simulink model "SimuNolineal"  (R2023b)
settings: Solver=VariableStepAuto  StartTime=0.0  StopTime=30  RelTol=1e-3
undefined symbols (not defined in the file): B, g, I, kd, ki, kp, kuf, kuf_0, lc, m, r
libraries: slpidlib x1
settings Model: Creator=sslan  LastModifiedBy=sslan

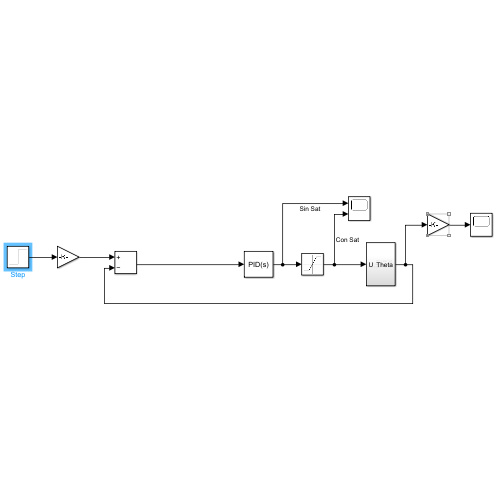
[thumbnail: Simulink's stored preview of the top-level diagram]
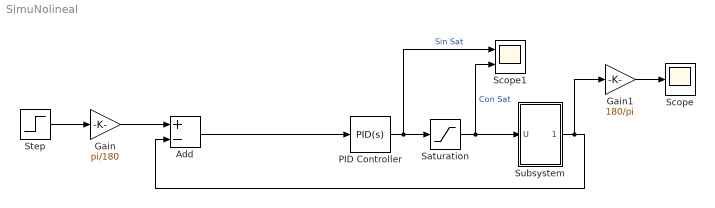
== system SimuNolineal ==
  Add : Sum  Inputs=+-
  Gain : Gain  Gain=pi/180
  Gain1 : Gain  Gain=180/pi
  PID Controller : slpidlib/PID Controller  Controller=PID  Form=Parallel  TimeDomain=Continuous-time  UseExternalTs=off  SampleTime=-1  IntegratorMethod=Forward Euler  FilterMethod=Forward Euler  ControllerParametersSource=internal  P=kp  I=ki  UseKiTs=off  D=kd  N=100  UseFilter=on  TunerSelectOption=Transfer Function Based (PID Tuner App)  InitialConditionSource=internal  InitialConditionForIntegrator=0  InitialConditionForFilter=0  DifferentiatorICPrevScaledInput=0  ExternalReset=none  TrackingMode=off  Kt=1  LimitOutput=off  SatLimitsSource=internal  UpperSaturationLimit=inf  LowerSaturationLimit=-inf  LinearizeAsGain=on  AntiWindupMode=none  Kb=1  LimitIntegrator=off  UpperIntegratorSaturationLimit=inf  LowerIntegratorSaturationLimit=-inf  POutMin=[]  POutMax=[]  IOutMin=[]  IOutMax=[]  DOutMin=[]  DOutMax=[]  NOutMin=[]  NOutMax=[]  SumOutMin=[]  SumOutMax=[]  SaturationOutMin=[]  SaturationOutMax=[]  PParamMin=[]  PParamMax=[]  IParamMin=[]  IParamMax=[]  DParamMin=[]  DParamMax=[]  NParamMin=[]  NParamMax=[]  KbParamMin=[]  KbParamMax=[]  KtParamMin=[]  KtParamMax=[]  KbOutMin=[]  KbOutMax=[]  KtOutMin=[]  KtOutMax=[]  IntegratorOutMin=[]  IntegratorOutMax=[]  FilterOutMin=[]  FilterOutMax=[]  SumI1OutMin=[]  SumI1OutMax=[]  SumI2OutMin=[]  SumI2OutMax=[]  SumI3OutMin=[]  SumI3OutMax=[]  SumI4OutMin=[]  SumI4OutMax=[]  SumDOutMin=[]  SumDOutMax=[]  DifferentiatorOutMin=[]  DifferentiatorOutMax=[]  FilterDiffOutCoefMin=[]  FilterDiffOutCoefMax=[]  ReciprocalOutMin=[]  ReciprocalOutMax=[]  SumDenOutMin=[]  SumDenOutMax=[]  SumNumOutMin=[]  SumNumOutMax=[]  DivideOutMin=[]  DivideOutMax=[]  UdiffTsProdOutMin=[]  UdiffTsProdOutMax=[]  NTsProdOutMin=[]  NTsProdOutMax=[]  UintegralTsProdOutMin=[]  UintegralTsProdOutMax=[]  UngainTsProdOutMin=[]  UngainTsProdOutMax=[]  ClampingZeroOutDataTypeStr=Inherit: Inherit via back propagation  ClampingZeroOutMin=[]  ClampingZeroOutMax=[]  FilterDenConstantOutDataTypeStr=Inherit: Inherit via back propagation  FilterDenConstantOutMin=[]  FilterDenConstantOutMax=[]  PCopyOutDataTypeStr=Inherit: Inherit via back propagation  PCopyOutMin=[]  PCopyOutMax=[]  NCopyOutDataTypeStr=Inherit: Inherit via back propagation  NCopyOutMin=[]  NCopyOutMax=[]  IntegratorContinuousStateAttributes=''  IntegratorStateMustResolveToSignalObject=off  IntegratorRTWStateStorageClass=Auto  FilterContinuousStateAttributes=''  FilterStateMustResolveToSignalObject=off  FilterRTWStateStorageClass=Auto  ParallelPVariant=InternalParameters  IdealPVariant=Disabled  IVariant=InternalParameters  DVariant=InternalParameters  IntegratorVariant=Continuous  SatVariant=Disabled  AWVariant=Passthrough  PCopyVariant=Disabled  TRVariant=Disabled  FdbkBlocksVariant=Forward  IdealPFdbkVariant=Disabled  SatFdbkVariant=Disabled  DerivativeFilterVariant=ContFilter  NVariant=InternalParameters  NCopyVariant=Disabled  FilterICVariant=InternalICsFilter  IntegratorICVariant=InternalICs  ExternalResetVariant=Disabled  TRSumVariant=Passthrough  SumFdbkVariant=Disabled  SumVariant=Sum_PID  TsampFilterVariant=InternalTs  TsampNgainVariant=Passthrough  TsampIntegralVariant=Disabled_SignalSpec  ExternalSaturationOutDataTypeStr=Inherit: Same as second input
  Saturation : Saturate  UpperLimit=100  LowerLimit=0
  Scope : Scope
  Scope1 : Scope  NumInputPorts=2
  Step : Step  After=145  SampleTime=0
  Subsystem : Subsystem
  wires:
  Subsystem/1(Theta) -> Gain1/1, Add/2
  Saturation/1 -> Scope1/2, Subsystem/1(U)  "Con Sat"
  PID Controller/1 -> Scope1/1, Saturation/1  "Sin Sat"
  Step/1 -> Gain/1
  Gain/1 -> Add/1
  Gain1/1 -> Scope/1
  Add/1 -> PID Controller/1

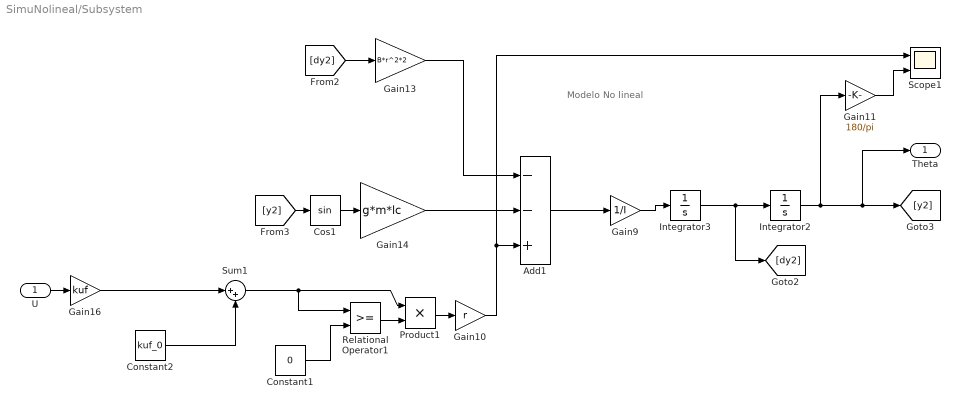
== system SimuNolineal/Subsystem ==
  note: Modelo No lineal
  U : Inport
  Add1 : Sum  Inputs=--+
  Constant1 : Constant  Value=0
  Constant2 : Constant  Value=kuf_0
  Cos1 : Trigonometry
  Gain10 : Gain  Gain=r
  Gain11 : Gain  Gain=180/pi
  Gain13 : Gain  Gain=B*r^2*2
  Gain14 : Gain  Gain=g*m*lc
  Gain16 : Gain  Gain=kuf
  Gain9 : Gain  Gain=1/I
  Integrator2 : Integrator
  Integrator3 : Integrator
  Product1 : Product
  Relational Operator1 : RelationalOperator  OutDataTypeStr=boolean  RndMeth=Simplest  InputSameDT=off
  Scope1 : Scope  NumInputPorts=2
  Sum1 : Sum  Inputs=|++
  Theta : Outport
  wires:
  Integrator2/1 -> Theta/1, [y2], Gain11/1
  [y2] -> Cos1/1
  Constant1/1 -> Relational Operator1/2
  Gain10/1 -> Add1/3, Scope1/1
  Relational Operator1/1 -> Product1/2
  Sum1/1 -> Product1/1, Relational Operator1/1
  Gain11/1 -> Scope1/2
  [dy2] -> Gain13/1
  Constant2/1 -> Sum1/2
  Gain14/1 -> Add1/2
  Gain13/1 -> Add1/1
  Gain16/1 -> Sum1/1
  Add1/1 -> Gain9/1
  Gain9/1 -> Integrator3/1
  Cos1/1 -> Gain14/1
  Integrator3/1 -> [dy2], Integrator2/1
  Product1/1 -> Gain10/1
  U/1 -> Gain16/1
